simulink model "squared_current"  (R2020b)
settings: Solver=ode15s  StartTime=0.0  StopTime=k*(Non+Noff)*Ts  FixedStep=Ts/100  RelTol=1e-3
undefined symbols (not defined in the file or in its folder): plecs
libraries: plecslib x2
settings Model: Creator=bente  LastModifiedBy=bente

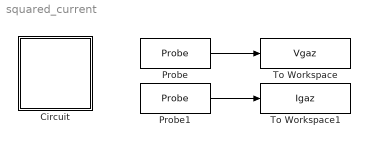
== system squared_current ==
  Circuit : Subsystem  LoadFcn=plecs('sl', 200);  InitFcn=plecs('sl', 214);  StartFcn=plecs('sl', 208);  StopFcn=plecs('sl', 209);  mask(PlecsCircuit){PLECSData=<binary blob, 4532 chars, not shown>}
      mask prompts: PLECSData "PLECS Data (Do not delete or modify!)"
      mask init:
      | % PLACE CUSTOM INITIALIZATIONS ABOVE
      | % DO NOT REMOVE
      | plecs('sl', 215);
      | % DO NOT REMOVE
      settings: CopyFcn=plecs('sl', 203);  DeleteFcn=plecs('sl', 205);  UndoDeleteFcn=plecs('sl', 206);  PreSaveFcn=plecs('sl', 211);  PostSaveFcn=plecs('sl', 201);  NameChangeFcn=plecs('sl', 210);  DestroyFcn=plecs('sl', 207);  PreCopyFcn=plecs('sl', 216);  OpenFcn=plecs('sl', 202);  ErrorFcn=plerrorfcn
      mask Help: web(['file:///' fullfile(plecsdoc, 'creatingacircuit.html')])
      mask Display: disp('PLECS\nCircuit')
  Probe : plecslib/Probe  tagno=1
      settings: SourceProductName=PLECS
  Probe1 : plecslib/Probe  tagno=2
      settings: SourceProductName=PLECS
  To Workspace : ToWorkspace  VariableName=Vgaz  SaveFormat=Timeseries  SampleTime=-1
  To Workspace1 : ToWorkspace  VariableName=Igaz  SaveFormat=Timeseries  SampleTime=-1
  wires:
  Probe/1 -> To Workspace/1
  Probe1/1 -> To Workspace1/1

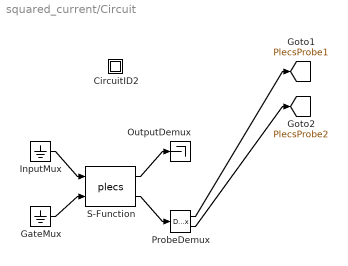
== system squared_current/Circuit ==
  " CircuitID2 " : Subsystem
  " GateMux " : Ground
  " InputMux " : Ground
  " OutputDemux " : Terminator
  " ProbeDemux " : Demux  Outputs=[ 1 1 ]
  " S-Function " : S-Function  FunctionName=plecs  SFunctionDeploymentMode=off  EnableBusSupport=off
  tag scope: PlecsProbe1=global, PlecsProbe2=global
  wires:
  " InputMux "/1 -> " S-Function "/1
  " GateMux "/1 -> " S-Function "/2
  " S-Function "/1 -> " OutputDemux "/1
  " S-Function "/2 -> " ProbeDemux "/1
  " ProbeDemux "/1 -> [PlecsProbe1]
  " ProbeDemux "/2 -> [PlecsProbe2]

== system squared_current/Circuit/ CircuitID2  ==
